simulink model "MMPT_CTRL"  (R2023a)
settings: Solver=FixedStepDiscrete  StartTime=0.0  StopTime=inf  FixedStep=1e-5  RelTol=1e-3  EnableMultiTasking=on
undefined symbols (not defined in the file or in its folder): Down, GPTRIP1SEL, TZ1, Up
libraries: c2802xlib x3, powerlib_extras x2
settings Model: ExtModeTrigDuration=8  Creator=Rahul  LastModifiedBy=dell
settings OptimizationCC: DefaultUnderspecifiedDataType=single  EnhancedBackFolding=on  PassReuseOutputArgsAs=Individual arguments  MaxStackSize=1024  OptimizeBlockOrder=speed  DifferentSizesBufferReuse=on  OptimizationCustomize=off  DenormalBehavior=FlushToZero  EfficientTunableParamExpr=on
settings DebuggingCC: ParameterTunabilityLossMsg=error  UnconnectedInputMsg=warning  UnconnectedOutputMsg=warning  UnconnectedLineMsg=warning
settings HardwareCC: ProdBitPerChar=16  ProdBitPerInt=16  ProdBitPerPointer=32  ProdBitPerSizeT=32  ProdBitPerPtrDiffT=32  ProdLargestAtomicInteger=Integer  ProdLargestAtomicFloat=None  ProdWordSize=16  ProdLongLongMode=on  ProdHWDeviceType=Texas Instruments->C2000  HardwareBoardFeatureSet=SoCBlockset
settings ModelReferenceCC: EnableRefExpFcnMdlSchedulingChecks=on  ModelReferenceNumInstancesAllowed=Single
settings SFSimCC: MATLABDynamicMemAlloc=off
settings RTWCC: Description=Embedded Coder  SystemTargetFile=ert.tlc  HardwareBoard=TI Delfino F28379D LaunchPad  TemplateMakefile=ert_default_tmf  Toolchain=Texas Instruments Code Composer Studio (C2000)  BuildConfiguration=Faster Runs  DLArmComputeVersion=19.05
settings CodeAppCC: ForceParamTrailComments=on  IgnoreCustomStorageClasses=off  OperatorAnnotations=on  SimulinkDataObjDesc=on  SFDataObjDesc=on  InsertBlockDesc=on
settings ERTTargetCC: CodeReplacementLibrary=TI C28x  SupportContinuousTime=on  ExtModeTransport=4  ExtModeStaticAlloc=on  ExtModeStaticAllocSize=10000  ExtModeMexFile=ext_xcp  ExtModeIntrfLevel=Level2 - Open

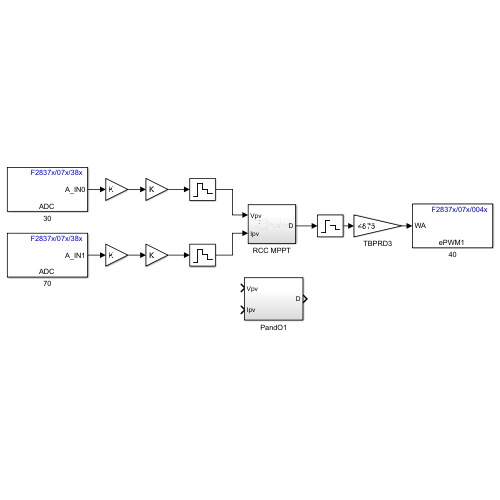
[thumbnail: Simulink's stored preview of the top-level diagram]
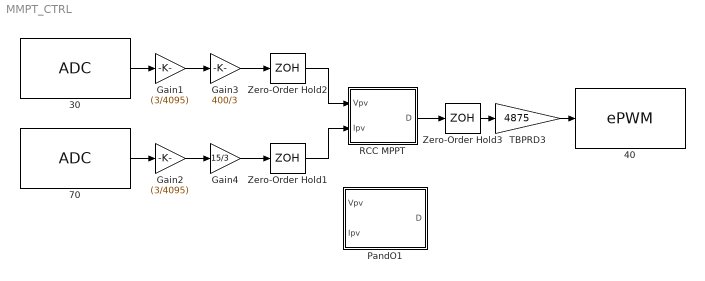
== system MMPT_CTRL ==
  30 : c2802xlib/ADC  blkParamProc=C2000_Type4  ADCModule=A  samplingMode=Single sample mode  ADCResolution=12-bit (Single-ended input)  useSOC1=SOC0  useSOC2=SOC0_SOC1  SOCAcquisitionWindow=15  SOCTriggerSource=Software  SOCInterruptTrigger=No ADCINT  Ts=1e-5  dType=double  postInterrupt=off  interruptSel=ADCINT1  ADCINTContinuous=on  endma=off  chdma=1  conv1=ADCINA0  conv2=ADCINA0 and ADCINB0  conv1_Type4=ADCIN0  conv2_Type4=ADCIN0 and ADCIN1
  40 : c2802xlib/ePWM  PwmType=C2000_Type4  useModule=ePWM1  ePWMxLINKTBPRD=Not Linked  periodUnits=Clock cycles  timerSource=Specify via dialog  timerPeriod_clk=4999  timerPeriod_sec=0.0001  tbshadow=Counter equals to zero  countingMode=Up-Down  phaseActiveEnable=Disable  phaseDirection=Count down after sync  phaseActive=0  synchronizationEnable=off  dcaevt1Sync=off  dcbevt1Sync=off  synchronizationOption=Disable  dcbevt1SyncOut=off  dcaevt1SyncOut=off  cmpdSyncOut=off  cmpcSyncOut=off  cmpbSyncOut=off  zeroSyncOut=off  swfSyncOut=off  perSynchronizationOption=Counter equals to period (CTR=PRD)  clockPrescale=1  HSclockPrescale=1  enswap=off  ePWMxAStatus=on  ePWMxAactionLogic1=Do nothing  ePWMxAactionLogic2=Do nothing  ePWMxAactionLogic3=Clear  ePWMxAactionLogic4=Set  ePWMxAactionLogic5=Do nothing  ePWMxAactionLogic6=Do nothing  ePWMxACSFenable=off  ePWMxACSFvalue=Forcing disable  ePWMxASFreload=Zero  ePWMxBStatus=off  ePWMxBactionLogic1=Do nothing  ePWMxBactionLogic2=Do nothing  ePWMxBactionLogic3=Clear  ePWMxBactionLogic4=Set  ePWMxBactionLogic5=Do nothing  ePWMxBactionLogic6=Do nothing  ePWMxBCSFenable=off  ePWMxBCSFvalue=Forcing disable  ePWMxBSFreload=Zero  ePWNxBOutWay=off  ePWMxLINKCMPA=Not Linked  CMPAUnits=Clock cycles  CMPASource=Input port  CMPAValue_per=50  CMPAValue_clk=0  enCMPAshadow=Counter equals to zero (CTR=Zero)  ePWMxLINKCMPB=Not Linked  CMPBUnits=Clock cycles  CMPBSource=Specify via dialog  CMPBValue_per=50  CMPBValue_clk=0  enCMPBshadow=Counter equals to zero (CTR=Zero)  ePWMxLINKCMPC=Not Linked  CMPCUnits=Clock cycles  CMPCSource=Specify via dialog  CMPCValue_per=50  CMPCValue_clk=0  enCMPCshadow=Counter equals to zero (CTR=Zero)  ePWMxLINKCMPD=Not Linked  CMPDUnits=Clock cycles  CMPDSource=Specify via dialog  CMPDValue_per=50  CMPDValue_clk=32000  enCMPDshadow=Counter equals to zero (CTR=Zero)  enableDBePWMxA=off  enableDBePWMxB=off  enhalfcycle=off  DBpolarity=Active high (AH)  DBedgeDelay=Positive  DBSource_ePWMxA=ePWMxB  DBSource_ePWMxB=ePWMxB  DBPeriodUnits=Clock cycles  DBperiodSource=Specify via dialog  REDperiod=7500  FEDperiod=7500  REDperiod_sec=0  FEDperiod_sec=0  LoadModeDBRED=Immediate without using shadow  LoadModeDBFED=Immediate without using shadow  adcstartModuleA=off  adcrequestEventA=First event  adcstartEventA=Digital Compare Module A Event 1 start of conversion (DCAEVT1.soc)  adcstartEventA_type2=Counter equals to zero (CTR=Zero)  adcstartModuleB=off  adcrequestEventB=First event  adcstartEventB=Counter equals to zero (CTR=Zero)  adcstartEventB_type2=Counter equals to zero (CTR=Zero)  intEn=off  intPrd=First event  intSel=Counter equals to zero (CTR=Zero)  intSel_type2=Counter equals to zero (CTR=Zero)  hrpe=off  enHRPWM=off  HRPWM_LoadMode=Counter equals to period (CTR=PRD)  HRPWM_CTLMode=Duty or Period control mode  HRPWM_EDGMode=Both edge  hrpeb=off  enHRPWMB=off  HRPWM_LoadModeB=Counter equals to zero (CTR=ZERO)  HRPWM_CTLModeB=Duty or Period control mode  HRPWM_EDGModeB=Both edge  enHRDBRED=off  enHRDBFED=off  enSFO=on  enautoconv=on  chopperEnable=off  chopperFrequency=1  chopperFirstwidth=1  chopperDuty=12.5%  tripZonesource=Specify via dialog  tzselOSHT1=off  tzselOSHT2=off  tzselOSHT3=off  tzselOSHDCAEV1=off  tzselOSHDCBEV1=off  tzselCBC1=off  tzselCBC2=off  tzselCBC3=off  tzselCBCDCAEV2=off  tzselCBCDCBEV2=off  tzselOSHT4=off  tzselOSHT5=off  tzselOSHT6=off  tzselCBC4=off  tzselCBC5=off  tzselCBC6=off  enTzOstIntr=off  enTzCbcIntr=off  enTzDCAEVT1Intr=off  enTzDCAEVT2Intr=off  enTzDCBEVT1Intr=off  enTzDCBEVT2Intr=off  ePWMxAforced=No action  ePWMxBforced=No action  DCAEVT1forced=No action  DCBEVT1forced=No action  DCAEVT2forced=No action  DCBEVT2forced=No action  dcah=Trip Zone 1 input (TZ1)  dcal=Trip Zone 2 input (TZ2)  dcbh=Trip Zone 1 input (TZ1)  dcbl=Trip Zone 2 input (TZ2)  dcah_type2=GPTRIP1SEL/(TZ1)  dcal_type2=GPTRIP1SEL/(TZ1)  dcbh_type2=GPTRIP1SEL/(TZ1)  dcbl_type2=GPTRIP1SEL/(TZ1)  gendcaevt1=Event disabled  gendcaevt2=Event disabled  gendcbevt1=Event disabled  gendcbevt2=Event disabled  dcaevt1src=DCAEVT1 with sync  dcaevt2src=DCAEVT2 with sync  dcbevt1src=DCBEVT1 with sync  dcbevt2src=DCBEVT2 with sync  pulsesel=Counter equals to zero (CTR=Zero)  blankinv=off  blankoffset=0  blankwidth=0  evsrcsel=Filtered version of DCAEVT1 (DCAEVT1FILT)  encape=off
      settings: LibrarySourceBlock=c2837xDlib/ePWM
  70 : c2802xlib/ADC  blkParamProc=C2000_Type4  ADCModule=A  samplingMode=Single sample mode  ADCResolution=12-bit (Single-ended input)  useSOC1=SOC1  useSOC2=SOC0_SOC1  SOCAcquisitionWindow=15  SOCTriggerSource=Software  SOCInterruptTrigger=No ADCINT  Ts=1e-5  dType=double  postInterrupt=off  interruptSel=ADCINT1  ADCINTContinuous=on  endma=off  chdma=1  conv1=ADCINA0  conv2=ADCINA0 and ADCINB0  conv1_Type4=ADCIN1  conv2_Type4=ADCIN0 and ADCIN1
  Gain1 : Gain  Gain=(3/4095)
  Gain2 : Gain  Gain=(3/4095)
  Gain3 : Gain  Gain=400/3
  Gain4 : Gain  Gain=15/3
  PandO1 : Subsystem
  RCC MPPT : Subsystem
  TBPRD3 : Gain  Gain=4875
  Zero-Order Hold1 : ZeroOrderHold  SampleTime=0.003
  Zero-Order Hold2 : ZeroOrderHold  SampleTime=0.003
  Zero-Order Hold3 : ZeroOrderHold  SampleTime=0.003
  wires:
  Zero-Order Hold2/1 -> RCC MPPT/1(Vpv)
  Zero-Order Hold1/1 -> RCC MPPT/2(Ipv)
  30/1 -> Gain1/1
  Gain1/1 -> Gain3/1
  Gain2/1 -> Gain4/1
  70/1 -> Gain2/1
  RCC MPPT/1(D) -> Zero-Order Hold3/1
  Gain3/1 -> Zero-Order Hold2/1
  Gain4/1 -> Zero-Order Hold1/1
  Zero-Order Hold3/1 -> TBPRD3/1
  TBPRD3/1 -> 40/1

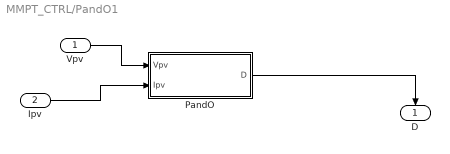
== system MMPT_CTRL/PandO1 ==
  Vpv : Inport
  Ipv : Inport  Port=2
  PandO : MATLAB Function  TreatAsAtomicUnit=on
  D : Outport
  wires:
  Ipv/1 -> PandO/2(Ipv)
  Vpv/1 -> PandO/1(Vpv)
  PandO/1(D) -> D/1

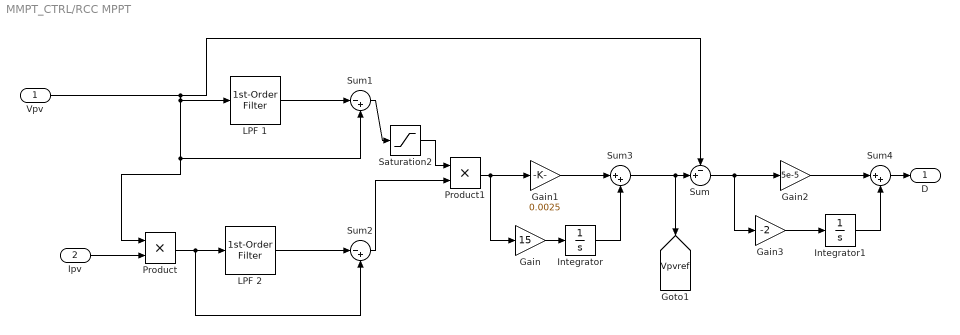
== system MMPT_CTRL/RCC MPPT ==
  Vpv : Inport
  Ipv : Inport  Port=2
  Gain : Gain  Gain=15
  Gain1 : Gain  Gain=0.0025
  Gain2 : Gain  Gain=5e-5
  Gain3 : Gain  Gain=-2
  Integrator : Integrator  UpperSaturationLimit=110  LowerSaturationLimit=70
  Integrator1 : Integrator  LimitOutput=on  UpperSaturationLimit=1  LowerSaturationLimit=-1
  LPF 1 : powerlib_extras/Control  Blocks/1st-Order  Filter  FilterType=Lowpass  Tc=1.25e-3  Initialize=on  Vac_Init=[80 0 100]  Vdc_Init=80  PlotResponse=off  param1=[0 500 1]
  LPF 2 : powerlib_extras/Control  Blocks/1st-Order  Filter  FilterType=Lowpass  Tc=1.25e-3  Initialize=on  Vac_Init=[80 0 100]  Vdc_Init=80  PlotResponse=off  param1=[0 500 1]
  Product : Product  RndMeth=Zero
  Product1 : Product  RndMeth=Zero
  Saturation2 : Saturate  UpperLimit=1  LowerLimit=-1
  Sum : Sum  Inputs=-+|
  Sum1 : Sum  Inputs=|-+
  Sum2 : Sum  Inputs=|-+
  Sum3 : Sum  Inputs=|++
  Sum4 : Sum  Inputs=|++
  D : Outport
  tag scope: Vpvref=global
  wires:
  Product/1 -> LPF 2/1, Sum2/2
  Gain/1 -> Integrator/1
  LPF 2/1 -> Sum2/1
  LPF 1/1 -> Sum1/1
  Sum2/1 -> Product1/2
  Integrator/1 -> Sum3/2
  Gain1/1 -> Sum3/1
  Ipv/1 -> Product/2
  Vpv/1 -> Sum/1, Sum1/2, Product/1, LPF 1/1
  Sum/1 -> Gain3/1, Gain2/1
  Gain2/1 -> Sum4/1
  Gain3/1 -> Integrator1/1
  Sum3/1 -> [Vpvref], Sum/2
  Integrator1/1 -> Sum4/2
  Sum1/1 -> Saturation2/1
  Product1/1 -> Gain/1, Gain1/1
  Saturation2/1 -> Product1/1
  Sum4/1 -> D/1

== matlab function MMPT_CTRL/PandO1/PandO ==
  data: D output; Vpv input; Ipv input

% f =10000 hz (G)
function D  = PandO(Vpv, Ipv)


Dinit = 0.7;  %Initial value for D output
Dmax = 0.85;   %Maximum value for D
Dmin = 0.65;   %Minimum value for D
deltaD = 0.005; %Increment value used to increase/decrease the duty cycle D


persistent Vold Pold Dold;

dataType = 'double';

if isempty(Vold)
    Vold=0;
    Pold=0;
    Dold=Dinit;
end
P= Vpv*Ipv;
dV= Vpv - Vold;
dP= P - Pold;

if dP ~= 0
    if dP < 0
        if dV < 0
            D = Dold - deltaD;
        else
            D = Dold + deltaD;
        end
    else
        if dV < 0
            D = Dold + deltaD;
        else
            D = Dold - deltaD;
        end    
    end
else
    D=Dold;
end

if D >= Dmax || D<= Dmin
    D=Dold;
end

Dold=D;
Vold=Vpv;
Pold=P;
